simulink model "Controller_damping_cbf"  (R2026b)
settings: Solver=ode4  StopTime=Inf  FixedStep=1e-3
values from neighbouring files (symbols this model uses):
  cbf_damping_params = [cbf_p_ths; cbf_v_ths; cbf_v_0; cbf_gamma; cbf_d_max;                        cbf_w_lin; cbf_w_quad; plane_normal; plane_offset;                        cbf_latch_entry; cbf_zone_hyst; cbf_latch_alpha; cbf_clip_drift;                        cbf_tau_rate; cbf_dt; cbf_gamma_pos_scale]    [init_damping_cbf.m]
  Dn = 20 * ones(7,1)    [init_damping_cbf.m]
  H_0_cy = H_0_pr * H_pr_cy    [init_damping_cbf.m]
  H_home = getTransform(Franka_robot, q_home, 'panda_link8', 'panda_link0')    [init_damping_cbf.m]
  Kn = 0 * ones(7,1)    [init_damping_cbf.m]
  q_home = q_init    [init_damping_cbf.m]
  q_init = [0 0  0  -(2/4)*pi  0  pi/2  -pi/4]'    [init_damping_cbf.m]
undefined symbols (not defined in the file or in its folder): DiscIntNeverNeededParam, Fext_mag, T_final, X, Y, Z
libraries: sm_lib x162, nesl_utility x44, matrix_library x3, Robotics_lib x1
(part 8 of 12)

== matlab function Controller_damping_cbf/Dynamic Parameters/Mass Matrix1 ==
  data: q_state input; M output
function M = Franka_MassmMatrix(q_state)
% Author: TU Wien, ACIN Robotics group
% Optimized and generated from Maple
% hier wurden
% M_rot := Matrix(M_rot, shape=symmetric):
% M := simplify(Matrix( simplify(M_trans) + simplify(M_rot), shape=symmetric)):
% ausgefuehrt 

  M = zeros(7,7);

  t378 = q_state(6);
  t364 = sin(t378);
  t379 = q_state(5);
  t365 = sin(t379);
  t377 = q_state(7);
  t370 = cos(t377);
  t337 = 0.12763550042100000000e-2 * t370;
  t363 = sin(t377);
  t317 = 0.51602752476000000000e-3 * t363;
  t532 = t317 + 0.27219646194675000000e-1;
  t504 = t337 + t532;
  t308 = 0.13614453378240000000e-2 * t363;
  t267 = 0.5826996021941340000e-3 - t308;
  t357 = t370 ^ 2;
  t600 = 0.15804348732630080000e-2 * t357;
  t93 = t267 + (0.48418875570424600000e-2 * t363 + 0.55042935974400000000e-3) * t370 - t600;
  t45 = t365 * t93 + t504;
  t872 = t45 * t364;
  t371 = cos(t378);
  t871 = t45 * t371;
  t380 = q_state(4);
  t373 = cos(t380);
  t271 = 0.60149e-1 * t371 + 0.14117e-1 * t364;
  t372 = cos(t379);
  t638 = 0.10517e-1 * t365;
  t411 = -t271 * t372 + t638;
  t826 = 0.825e-1 + t411;
  t846 = t373 * t826;
  t381 = q_state(3);
  t367 = sin(t381);
  t474 = -0.10517e-1 * t370 - 0.4252e-2 * t363;
  t240 = -t474 + 0.88e-1;
  t639 = 0.61597e-1 * t364;
  t403 = t240 * t371 + t639;
  t812 = t365 * t403;
  t475 = 0.10517e-1 * t363 - 0.4252e-2 * t370;
  t844 = t372 * t475;
  t853 = (t844 - t812) * t367;
  t316 = 0.54835910640823200000e-3 * t363;
  t559 = 0.16724826617837780000e-2 * t370;
  t580 = 0.26431758938496000000e-1 * t364;
  t423 = t559 + t580;
  t311 = 0.10967182128164640000e-2 * t363;
  t553 = 0.33449653235675560000e-2 * t370;
  t442 = 0.11022068765350630000e-1 + t553;
  t183 = -t311 + t442;
  t358 = t371 ^ 2;
  t753 = t183 * t358;
  t642 = t316 - t423 - 0.44842466056464210000e-2 + t753;
  t250 = 0.12009367848960000000e-2 * t363 + 0.63347540234880000000e-1;
  t554 = 0.29704261916160000000e-2 * t370;
  t176 = t250 + t554;
  t351 = t363 ^ 2;
  t300 = 0.13297872941088000000e-4 * t351;
  t315 = 0.55042935974400000000e-3 * t363;
  t534 = -t315 - 0.57804776249276620000e-2;
  t333 = 0.24076459055801420000e-2 * t357;
  t592 = 0.79021743663150400000e-3 * t363;
  t721 = (-0.13614453378240000000e-2 + t592) * t370;
  t856 = t333 + t721;
  t833 = t534 + t856;
  t60 = -t300 + t833;
  t40 = -t364 * t60 + t176;
  t770 = t40 * t371;
  t870 = t642 - t770;
  t385 = -t365 * t475 - t372 * t403;
  t383 = q_state(1);
  t369 = sin(t383);
  t869 = t369 ^ 2;
  t376 = cos(t383);
  t868 = t376 ^ 2;
  t867 = t373 - 0.1e1;
  t313 = 0.68072266891200000000e-3 * t363;
  t222 = (0.24209437785212300000e-2 * t363 + 0.27521467987200000000e-3) * t370;
  t601 = 0.79021743663150400000e-3 * t357;
  t839 = t222 - t601;
  t413 = -0.29134980109706700000e-3 - t839;
  t87 = t313 + t413;
  t76 = t365 * t87;
  t834 = t315 + 0.32797153116247448000e-1 - t721;
  t481 = -t333 + t834;
  t62 = t300 + t481;
  t866 = t62 * t373;
  t65 = -0.825e-1 - t385;
  t865 = t65 * t373;
  t864 = t87 * t364;
  t74 = t87 * t371;
  t713 = t364 * t365;
  t863 = t87 * t713;
  t585 = 0.33449653235675560000e-2 * t363;
  t190 = 0.10967182128164639999e-2 * t370 + t585 + 0.18713819462921000000e-3;
  t144 = t190 * t365;
  t99 = 0.11357396418885000000e-1 - t144;
  t862 = t99 * t364;
  t673 = t300 + t315;
  t54 = (-0.69751885789075550000e-2 - t673 + t856) * t358;
  t710 = t364 * t371;
  t658 = t183 * t710;
  t817 = t658 - t54;
  t348 = 0.61597e-1 * t371;
  t836 = t240 * t364 - t348;
  t125 = 0.384e0 + t836;
  t366 = sin(t380);
  t848 = t125 * t366;
  t449 = 0.98827089590400000000e-3 * t363 + 0.52129746651620000000e-1;
  t556 = 0.24444132201840000000e-2 * t370;
  t198 = t449 + t556;
  t861 = t198 * t371;
  t182 = 0.59408523832320000000e-2 * t370 + 0.24018735697920000000e-2 * t363 + 0.12669508046976000000e0;
  t329 = 0.48152918111602840020e-2 * t357;
  t299 = 0.26595745882176000000e-4 * t351;
  t310 = 0.11008587194880000000e-2 * t363;
  t674 = t299 + t310;
  t508 = 0.11560955249855324002e-1 + t674;
  t590 = 0.15804348732630079999e-2 * t363;
  t722 = (-0.27228906756480000000e-2 + t590) * t370;
  t788 = t722 + t329 - t508;
  t645 = t364 * t788 - t182;
  t860 = t371 * t645;
  t334 = 0.15804348732630079999e-2 * t357;
  t521 = -t334 + t267;
  t724 = (0.48418875570424600020e-2 * t363 + 0.55042935974400000000e-3) * t370;
  t488 = t724 + t521;
  t859 = t488 * t365;
  t705 = t365 * t372;
  t560 = 0.14820000000000000000e-2 * t370;
  t287 = t364 * t560;
  t587 = 0.23920000000000000000e-2 * t363;
  t716 = (0.68200e-3 + t587) * t364;
  t451 = 0.17120000000000000000e-2 * t357 + 0.14600000000000000000e-2;
  t714 = t363 * t370;
  t517 = 0.49780000000000000000e-2 * t714;
  t394 = -t451 + t517;
  t762 = t394 * t371;
  t784 = t762 - t716 - t287 - 0.42340e-2;
  t858 = t705 * t784;
  t133 = t504 * t371;
  t824 = 0.11357396418885000000e-1 * t364 - 0.24178658687700000000e-2;
  t797 = t133 + t824;
  t79 = t797 * t372;
  t359 = t372 ^ 2;
  t427 = 0.10967182128164640000e-2 * t370 + t585;
  t189 = t427 + 0.18713819462921000000e-3;
  t748 = t189 * t364;
  t606 = t748 + 0.5437511053345940e-2;
  t849 = t93 * t371;
  t815 = t849 - t606;
  t857 = t815 * t359;
  t598 = 0.24890000000000000000e-2 * t357;
  t416 = t598 + 0.85600000000000000000e-3 * t714;
  t38 = t849 - t748 - 0.54375110533459400000e-2;
  t185 = -0.59408523832320000000e-2 * t363 + 0.47796540830203740000e-1 + 0.24018735697920000000e-2 * t370;
  t752 = t185 * t365;
  t540 = t752 + 0.27752814537092170000e0;
  t854 = -t371 * t99 + t540;
  t352 = t364 ^ 2;
  t284 = t370 * t592;
  t495 = t284 + 0.24209437785212300000e-2 * t357;
  t759 = (t495 + 0.1194710953979893e-2) * t352;
  t852 = 0.25054324779447817000e-1 + t759;
  t382 = q_state(2);
  t375 = cos(t382);
  t850 = t375 ^ 2;
  t847 = t826 * t366;
  t256 = 0.56786982094425000000e-2 * t364 - 0.12089329343850000000e-2;
  t229 = t256 * t373;
  t845 = t366 * t371;
  t374 = cos(t381);
  t700 = t366 * t374;
  t694 = t367 * t374;
  t688 = t371 * t373;
  t687 = t371 * t374;
  t683 = t373 * t374;
  t468 = 0.39252e-1 * t367 - 0.27518e-1 * t374;
  t843 = t375 * t468;
  t581 = 0.21751134959804000000e-1 * t364;
  t842 = (t581 - 0.46305794820080000000e-2 + t861) * t372;
  t672 = 0.31608697465260159998e-2 * t357 + 0.27228906756480000000e-2 * t363;
  t461 = (0.96837751140849200040e-2 * t363 + 0.11008587194880000000e-2) * t370 - t672 + 0.11653992043882680000e-2;
  t72 = t461 * t371;
  t804 = t504 * t364;
  t158 = t416 + 0.28220000000000000000e-2;
  t763 = t158 * t358;
  t389 = t763 + t416 - 0.27050000000000000000e-2;
  t307 = 0.14820000000000000000e-2 * t363;
  t558 = 0.23920000000000000000e-2 * t370;
  t491 = -t307 + t558;
  t657 = (0.21800000000000000000e-3 + t491) * t710;
  t841 = (-t657 + t389) * t359;
  t332 = 0.24076459055801420010e-2 * t357;
  t593 = 0.79021743663150399997e-3 * t363;
  t838 = -(-0.13614453378240000000e-2 + t593) * t370 - t332 + t673;
  t53 = (0.69751885789075550010e-2 + t838) * t358;
  t285 = t370 * t593;
  t837 = t285 + 0.25022978729410880010e-2 * t357;
  t298 = 0.81354094419858000000e-4 * t351;
  t318 = 0.11947109539798930000e-2 * t352;
  t670 = t318 - t298;
  t579 = 0.61597000000000000000e-1 * t364;
  t216 = 0.10517000000000000000e-1 * t363 - 0.42520000000000000000e-2 * t370;
  t197 = 0.10517000000000000000e-1 * t370 + 0.42520000000000000000e-2 * t363 + 0.88000000000000000000e-1;
  t742 = t197 * t371;
  t681 = -t216 * t365 - t372 * t742;
  t835 = -t372 * t579 + t681 + 0.82500000000000000000e-1;
  t473 = 0.60149e-1 * t364 - 0.14117e-1 * t371;
  t234 = t473 + 0.384e0;
  t728 = t234 * t373;
  t832 = t366 * t411 - t728;
  t342 = 0.13297872941088e-4 * t351;
  t67 = -t342 + t833;
  t57 = t67 * t364;
  t831 = t57 - 0.1e1 * t176;
  t415 = 0.49780000000000000000e-2 * t357 + 0.17120000000000000000e-2 * t714;
  t167 = 0.5644000000000000000e-2 + t415;
  t122 = t167 * t358;
  t492 = -0.47840000000000000000e-2 * t370 + 0.29640000000000000000e-2 * t363;
  t210 = 0.43600e-3 - t492;
  t126 = t210 * t710;
  t680 = t122 - t126;
  t830 = 0.31784000000000000000e-1 + t680 - 0.1e1 * t416;
  t314 = 0.63817750210500000000e-3 * t363;
  t567 = 0.25801376238000000000e-3 * t370;
  t445 = 0.55993270925625000000e-2 + t567;
  t191 = -t314 + t445;
  t676 = t284 + 0.25022978729410880000e-2 * t357;
  t84 = 0.25565950283854690000e-2 - t676 + t670;
  t33 = t84 + t817;
  t829 = t33 * t365 - 0.1e1 * t191;
  t828 = -0.1e1 * t185 - 0.1e1 * t190 * t371;
  t368 = sin(t382);
  t171 = t368 * t468 + 0.249498e0 * t375;
  t572 = 0.21751134959804000000e-1 * t366;
  t825 = t133 - 0.24178658687700000000e-2;
  t823 = 0.56786982094425000000e-2 * t371 + 0.12908973617152500000e-1;
  t259 = 0.11357396418885000000e-1 * t366 - 0.52863517876992000000e-1;
  t309 = 0.12763550042100000000e-2 * t363;
  t566 = 0.51602752476000000000e-3 * t370;
  t444 = 0.11198654185125000000e-1 + t566;
  t175 = -t309 + t444;
  t756 = t175 * t365;
  t822 = (-t366 * t504 + t182) * t364 + 0.16910953236199946500e0 + t259 * t371 + (-0.1e1 * t756 + t79 - 0.31476782229750000000e-1) * t373 - 0.10663433246449500000e0 * t366;
  t589 = 0.15804348732630080000e-2 * t363;
  t813 = t364 * ((-0.27228906756480000000e-2 + t589) * t370 + 0.48152918111602840000e-2 * t357 - t674 - 0.11560955249855324000e-1);
  t37 = (-t182 + t813) * t371;
  t552 = 0.66899306471351120000e-2 * t370;
  t424 = -0.21934364256329280000e-2 * t363 + t552;
  t319 = 0.52863517876992000000e-1 * t364;
  t453 = 0.8968493211292842000e-2 + t553;
  t437 = t319 + t453;
  t408 = -(t424 + 0.22044137530701260000e-1) * t358 - t311 + t437;
  t97 = t189 * t365 - 0.11357396418885000000e-1;
  t771 = t371 * t97;
  t819 = (t37 - t408) * t372 + t771;
  t173 = t271 * t365 + 0.10517e-1 * t372;
  t406 = t173 * t367;
  t215 = t234 * t366;
  t207 = -0.825e-1 + t215;
  t803 = t207 + t846;
  t818 = t374 * t803 + t406;
  t263 = 0.25801376238000000000e-3 * t363 + 0.13609823097337500000e-1;
  t564 = 0.63817750210500000000e-3 * t370;
  t199 = t263 + t564;
  t739 = t199 * t373;
  t293 = 0.88e-1 * t364 + 0.384e0;
  t814 = t293 * t367;
  t338 = 0.98827089590400000000e-3 * t370;
  t448 = 0.24444132201840000000e-2 * t363 - 0.21447119530300000000e-1;
  t800 = -t338 + t448;
  t807 = t800 * t367;
  t628 = 0.345563e0 * t373;
  t472 = 0.41065e-1 * t365 + 0.11953e-1 * t372;
  t235 = t472 + 0.825e-1;
  t727 = t235 * t366;
  t502 = -t628 + t727;
  t806 = (t502 - 0.316e0) * t375;
  t805 = (-0.41065e-1 * t372 + 0.11953e-1 * t365) * t367;
  t345 = 0.345563e0 * t366;
  t290 = -0.825e-1 + t345;
  t726 = t235 * t373;
  t524 = t290 + t726;
  t105 = t524 * t374;
  t150 = t199 * t371;
  t802 = t256 + t150;
  t277 = t307 - 0.829200e-2;
  t659 = t167 * t710;
  t732 = t210 * t358;
  t801 = t277 - t558 + t659 + t732;
  t426 = -t560 - t587;
  t730 = (-t426 + 0.68200e-3) * t371;
  t799 = t394 * t364 + t730 - 0.45800e-3;
  t798 = t300 - 0.1e1 * t333 - 0.26431758938496000000e-1 * t371 + t834;
  t796 = 0.46331267916800000000e-2 - t837;
  t794 = 0.53124178491565338000e0 + t673 + 0.2251687828321245e-2 * t359;
  t618 = 0.7735484874e-2 * t370;
  t793 = 0.3127439544e-2 * t363 + t618;
  t660 = t158 * t710;
  t211 = 0.21800e-3 + t491;
  t731 = t211 * t358;
  t791 = -t660 - t731;
  t460 = -t670 + t837;
  t312 = 0.10967182128164639999e-2 * t363;
  t184 = -t312 + t442;
  t662 = t184 * t710;
  t790 = t662 - t460 + 0.48082828567067140000e-2;
  t484 = -t722 + 0.13950377157815110002e-1 + t674;
  t392 = -t739 + t199;
  t164 = t333 + t284 - 0.9457555763200000000e-3;
  t787 = t164 * t358 - t658;
  t565 = 0.54835910640823200000e-3 * t370;
  t588 = 0.16724826617837780000e-2 * t363;
  t430 = t565 + t588;
  t202 = t430 + 0.9356909731460500000e-4;
  t737 = t202 * t371;
  t786 = t864 - 0.1e1 * t737;
  t341 = 0.4815291811160284002e-2 * t357;
  t678 = t722 + t341;
  t785 = -0.1e1 * t319 + ((-t508 + t678) * t364 - t182) * t371;
  t282 = t370 * t589;
  t336 = 0.13614453378240000000e-2 * t370;
  t671 = t315 + t336;
  t755 = (0.60427308755286430000e-2 + t671) * t352;
  t783 = t282 + t756 - 0.1e1 * t755;
  t782 = -t716 - 0.15700e-2;
  t489 = -t316 + t559;
  t186 = t489 + 0.44842466056464210000e-2;
  t326 = 0.56786982094425000000e-2 * t366;
  t528 = t326 - 0.21751134959804000000e-1;
  t545 = 0.26431758938496000000e-1 * t373;
  t573 = 0.12089329343850000000e-2 * t366;
  t780 = (t186 * t373 + (-0.1e1 * t528 + t545) * t364 + t573 - 0.46305794820080000000e-2) * t372 + t852 * t366;
  t156 = -0.85600000000000000000e-3 * t357 + 0.24890000000000000000e-2 * t714 - 0.73000000000000000000e-3;
  t709 = t364 * t372;
  t779 = -t156 * t709 - 0.86410e-2;
  t734 = (0.6042730875528643e-2 + t671) * t352;
  t777 = t734 + 0.65337013765020712700e0;
  t283 = t370 * t590;
  t353 = t365 ^ 2;
  t320 = 0.22516878283212450000e-2 * t353;
  t531 = t320 - 0.54359965714773641100e0;
  t754 = t182 * t364;
  t775 = 0.48418875570424600020e-2 * t357 + (t184 * t364 + 0.52863517876992000000e-1) * t371 + t283 + t531 - t754 - t755 + t756;
  t774 = -t176 * t372 + 0.56786982094425000000e-2;
  t773 = t870 * t365;
  t86 = t334 - t724 - 0.58269960219413400000e-3 + t308;
  t772 = t371 * t86;
  t537 = t197 * t364 + 0.38400000000000000000e0;
  t767 = (-t348 + t537) * t366;
  t766 = (-t199 + 0.21751134959804000000e-1 * t372) * t373;
  t523 = 0.6029433002587555e-2 + t671;
  t765 = (t300 + t523) * t358;
  t764 = (-0.99560000000000000000e-2 * t714 + 0.34240000000000000000e-2 * t357 + 0.29200000000000000000e-2) * t371;
  t121 = (0.2489553776598930000e-3 + t495) * t358;
  t758 = t800 * t365;
  t757 = t800 * t373;
  t137 = t176 * t366;
  t306 = 0.21934364256329279998e-2 * t363;
  t441 = 0.22044137530701260000e-1 + t552;
  t181 = -t306 + t441;
  t134 = t181 * t358;
  t187 = 0.69884864518486430000e-2 + t671;
  t751 = t187 * t373;
  t303 = 0.29704261916160000000e-2 * t363;
  t561 = 0.12009367848960000000e-2 * t370;
  t443 = 0.23898270415101870000e-1 + t561;
  t188 = -t303 + t443;
  t750 = t188 * t365;
  t749 = t188 * t373;
  t746 = t191 * t365;
  t745 = t191 * t366;
  t323 = 0.82500000000000000002e-1 * t366;
  t194 = t323 - 0.31600000000000000000e0 * t373 - 0.38400000000000000000e0;
  t744 = t194 * t371;
  t196 = 0.48888264403680000000e-2 * t370 + 0.19765417918080000000e-2 * t363 + 0.10425949330324000000e0;
  t743 = t196 * t364;
  t147 = t198 * t364;
  t741 = t198 * t373;
  t740 = t199 * t364;
  t149 = t199 * t366;
  t154 = t202 * t364;
  t738 = t202 * t365;
  t736 = t202 * t374;
  t490 = -t311 + t553;
  t203 = 0.11022068765350630e-1 + t490;
  t735 = t203 * t358;
  t205 = 0.187138194629210e-3 + t427;
  t733 = t205 * t365;
  t563 = 0.74100000000000000000e-3 * t370;
  t591 = 0.11960000000000000000e-2 * t363;
  t429 = -t563 - t591;
  t213 = -t429 + 0.34100e-3;
  t729 = t213 * t371;
  t723 = (0.68200000000000000000e-3 + t587) * t364;
  t254 = t314 - 0.55993270925625000000e-2;
  t720 = t254 * t366;
  t264 = 0.11198654185125000000e-1 - t309;
  t719 = t264 * t365;
  t718 = (0.4841887557042460002e-2 * t363 + 0.55042935974400000000e-3) * t370;
  t715 = t353 * t364;
  t712 = t364 * t366;
  t711 = t364 * t367;
  t708 = t364 * t373;
  t707 = t365 * t366;
  t706 = t365 * t371;
  t704 = t365 * t375;
  t703 = t366 * t367;
  t702 = t366 * t372;
  t701 = t366 * t373;
  t699 = t366 * t375;
  t698 = t367 * t365;
  t697 = t367 * t369;
  t696 = t367 * t372;
  t695 = t367 * t373;
  t692 = t367 * t376;
  t691 = t368 * t369;
  t690 = t368 * t376;
  t689 = t369 * t374;
  t686 = t371 * t375;
  t685 = t372 * t373;
  t684 = t372 * t375;
  t682 = t373 * t375;
  t656 = t211 * t710;
  t679 = t656 - t763;
  t344 = 0.3507900e-3 * t365;
  t288 = -0.925496e-3 - t344;
  t677 = t288 * t373 + t344;
  t647 = 0.825e-1 * t374;
  t295 = t368 * t647;
  t649 = 0.825e-1 * t366;
  t675 = -t375 * t649 - t295;
  t669 = t762 - 0.1e1 * t287;
  t666 = t373 * t759;
  t180 = -0.21934364256329279999e-2 * t363 + t441;
  t665 = t180 * t710;
  t664 = t181 * t710;
  t111 = t183 * t708;
  t663 = t374 * t753;
  t661 = t359 * t699;
  t655 = t365 * t699;
  t653 = t183 * t712;
  t652 = t366 * t686;
  t350 = 0.316e0 * t368;
  t651 = t368 * t649 + t647 * t682 - t350;
  t648 = 0.825e-1 * t367;
  t643 = -0.7850e-3 + (-0.34100e-3 - t591) * t364;
  t637 = 0.27454e-1 * t367;
  t631 = 0.249498e0 * t368;
  t630 = 0.735522e0 * t371;
  t623 = 0.384e0 * t699 * t374 + t651;
  t622 = 0.8676525e-3 * t365;
  t620 = 0.3127439544e-2 * t365;
  t619 = 0.7735484874e-2 * t365;
  t617 = 0.3127439544e-2 * t373;
  t616 = 0.7735484874e-2 * t373;
  t615 = 0.3127439544e-2 * t370;
  t614 = 0.735522e0 * t700;
  t613 = 0.6381775021050e-3 * t366;
  t612 = 0.2580137623800e-3 * t367;
  t611 = 0.6381775021050e-3 * t367;
  t609 = t728 - t847;
  t438 = t312 - t453;
  t604 = t438 * t365 + 0.3288975154738540000e-2;
  t603 = t79 - 0.80863245317250000000e-1;
  t602 = 0.23894219079597860000e-2 * t352;
  t596 = 0.50045957458821760020e-2 * t357;
  t595 = 0.28220000000000000000e-2 * t358;
  t594 = 0.74100000000000000000e-3 * t363;
  t586 = 0.31608697465260159998e-2 * t363;
  t584 = 0.66899306471351120000e-2 * t363;
  t583 = 0.49096519673609460000e-2 * t364;
  t578 = 0.88000000000000000000e-1 * t364;
  t577 = 0.24178658687700000000e-2 * t365;
  t576 = 0.49096519673609460000e-2 * t365;
  t575 = 0.26431758938496000000e-1 * t365;
  t574 = 0.54835910640823200000e-3 * t366;
  t570 = 0.31600000000000000000e0 * t366;
  t569 = 0.16724826617837780000e-2 * t367;
  t568 = 0.46305794820080000000e-2 * t367;
  t562 = 0.11960000000000000000e-2 * t370;
  t555 = 0.29640000000000000000e-2 * t370;
  t551 = 0.16724826617837780000e-2 * t371;
  t550 = 0.11357396418885000000e-1 * t371;
  t549 = 0.54835910640823200000e-3 * t373;
  t548 = 0.16724826617837780000e-2 * t373;
  t547 = 0.49096519673609460000e-2 * t373;
  t546 = 0.21751134959804000000e-1 * t373;
  t543 = 0.21751134959804000000e-1 * t371;
  t542 = t364 * t612;
  t541 = t364 * t611;
  t538 = t190 * t364 + 0.54375110533459400000e-2;
  t536 = t287 + 0.42340000000000000000e-2;
  t530 = 0.43502269919608000000e-1 * t366 - 0.11357396418885000000e-1;
  t529 = -t326 + 0.26431758938496000000e-1;
  t527 = 0.12089329343850000000e-2 * t867;
  t343 = 0.13297872941088e-4 * t357;
  t526 = -t343 - 0.11947109539798930000e-2;
  t525 = 0.23898270415101870000e-1 - t303;
  t522 = t540 + t872;
  t470 = -0.104419e0 * t366 - 0.5317e-1 * t373;
  t236 = -t470 - 0.825e-1;
  t520 = t236 * t374 - t637;
  t516 = t365 * t581;
  t515 = t364 * t549;
  t514 = t364 * t548;
  t513 = 0.49096519673609460000e-2 * t845;
  t512 = t364 * t563;
  t511 = t372 * t547;
  t503 = 0.48082828567067140000e-2 - t676;
  t501 = -0.52863517876992000000e-1 * t371 + t754;
  t425 = -0.21934364256329279998e-2 * t370 - t584;
  t201 = -t425 + 0.3742763892584200000e-3;
  t499 = -t201 * t364 - 0.10875022106691880000e-1;
  t498 = -0.56786982094425000000e-2 + t738;
  t266 = 0.9356909731460500000e-4 + t588;
  t496 = t266 + t565;
  t494 = -t284 - t598;
  t493 = -t285 - 0.24209437785212300010e-2 * t357;
  t487 = t504 + t859;
  t486 = -t565 - 0.1e1 * t266;
  t479 = -t298 + t503;
  t217 = -0.41065000000000000000e-1 * t372 + 0.11953000000000000000e-1 * t365;
  t478 = t217 * t374 + t367 * t524;
  t469 = -0.104419e0 * t373 + 0.5317e-1 * t366;
  t467 = -0.39252e-1 * t374 - 0.27518e-1 * t367;
  t466 = t496 * t365;
  t464 = (0.13297872941088000000e-4 * t357 - t670 - t817 - 0.46331267916800000000e-2) * t359 + t38 * t705 + t501;
  t463 = -0.1e1 * t318 - t479;
  t459 = t54 - t84;
  t328 = 0.48418875570424600000e-2 * t357;
  t456 = -t79 + t658 - t121 + (t494 + 0.175156065026714e-3) * t359 + t320 + t328 - 0.37693495392476464200e0;
  t253 = -t313 + 0.29134980109706700000e-3;
  t455 = -0.1e1 * t222 + t601 - 0.1e1 * t253;
  t454 = -0.5437511053345940e-2 * t365 - 0.24178658687700000000e-2;
  t260 = 0.56786982094425000000e-2 * t867;
  t446 = -0.54375110533459400000e-2 * t365 - 0.24178658687700000000e-2;
  t232 = 0.16724826617837780000e-2 * t374 + 0.988270895904e-3 * t367;
  t440 = 0.2444413220184e-2 * t367 + 0.54835910640823200000e-3 * t374;
  t439 = 0.7902174366315040000e-3 * t357 + t313 - 0.2913498010970670000e-3;
  t436 = (t469 - 0.316e0) * t375;
  t433 = 0.48888264403680000000e-2 * t363 - 0.19765417918080000000e-2 * t370 - 0.42894239060600000000e-1;
  t431 = -0.1e1 * t338 + t448;
  t428 = t562 - t594;
  t422 = -t546 + t326;
  t421 = t134 + t438;
  t231 = t263 * t366;
  t324 = 0.82500000000000000000e-1 * t366;
  t257 = t324 - 0.38400000000000000000e0;
  t420 = t257 * t618 + t231 - t250;
  t297 = 0.16270818883971600000e-3 * t351;
  t419 = t283 + t297 - 0.51131900567709380000e-2 - t602;
  t417 = -0.1e1 * t303 - t864 + t443;
  t172 = -t631 + t843;
  t409 = t366 * t472 - t628;
  t206 = -t430 - 0.93569097314605e-4;
  t402 = t423 + 0.4484246605646421e-2;
  t258 = -t324 + 0.31600000000000000000e0;
  t401 = t258 * t618 + t449;
  t400 = t430 + 0.935690973146050000e-4;
  t398 = -0.25527100084200000000e-2 * t370 - 0.10320550495200000000e-2 * t363 - 0.54439292389350000000e-1;
  t397 = 0.11881704766464000000e-1 * t370 + 0.48037471395840000000e-2 * t363 + 0.25339016093952000000e0;
  t396 = -t415 + 0.5410000000000000000e-2;
  t393 = -t415 + 0.33106000000000000000e-1;
  t390 = t602 + t665 - 0.1e1 * t283 - 0.1e1 * t297 - t596;
  t388 = t763 + t393;
  t386 = -t186 + 0.46305794820080000000e-2 * t373 - t573;
  t384 = -t125 * t373 + t366 * t385;
  t361 = t374 ^ 2;
  t360 = t373 ^ 2;
  t355 = t367 ^ 2;
  t354 = t366 ^ 2;
  t340 = 0.21751134959804000000e-1 * t374;
  t327 = 0.54835910640823200000e-3 * t367;
  t322 = 0.56786982094425000000e-2 * t365;
  t321 = 0.17515606502671400000e-3 * t353;
  t289 = t622 - 0.374176e-3;
  t286 = t367 * t567;
  t278 = 0.414600e-2 - t594;
  t276 = 0.47840000000000000000e-2 * t363 + 0.136400e-2;
  t274 = -0.2872e-1 * t375 - 0.3141e-2 * t368;
  t269 = t289 * t373;
  t261 = -0.82500000000000000002e-1 + t570;
  t255 = 0.38400000000000000000e0 + t578;
  t230 = t449 * t367;
  t228 = t256 * t366;
  t195 = 0.38400000000000000000e0 * t373 - t323 + 0.31600000000000000000e0;
  t193 = -t260 - 0.26431758938496000000e-1 * t366;
  t163 = t332 + t285 - 0.9457555763200000010e-3;
  t155 = t202 * t372;
  t145 = t191 * t373;
  t140 = t186 * t366;
  t129 = t433 * t365;
  t120 = t202 * t688;
  t106 = t154 + 0.6624110552949070e-2;
  t103 = -t194 + t578;
  t101 = -t190 + 0.11357396418885000000e-1 * t365;
  t90 = -t804 + t550 - 0.28391278634449500000e0;
  t89 = -0.61597000000000000000e-1 * t371 + t537;
  t77 = t87 * t374;
  t71 = -t489 * t364 + (-0.680722668912e-3 * t370 - 0.275214679872e-3 * t363 - 0.49096519673609460000e-2) * t371;
  t70 = t87 * t708;
  t68 = -t805 + t105;
  t51 = t844 + (-t639 - t742) * t365;
  t49 = -t372 * t639 + t681 + 0.825e-1;
  t42 = t371 * t496 - t864;
  t36 = -t656 + t389;
  t26 = 0.155920e-1 + t801 * t372 + t799 * t365;
  t25 = t429 * t372 + (t371 * t428 - t583 - t793 * (t293 - t348)) * t365 + (0.7735484874e-2 * t363 - t615) * (-(-0.384e0 * t371 + 0.61597e-1) * t372 + 0.825e-1 * t364);
  t24 = t798 * t372 + t74 * t365 - t150 + (t466 - t774) * t364;
  t20 = -t773 + (t188 + t737 - t864) * t372;
  t19 = ((t293 * t793 - t371 * t489 + t583) * t372 + (0.28244044800000000000e0 * t216 * t371 - t430) * t365) * t366 - 0.606805650e-1 * t474 * t867 * t372 + (-0.1e1 * t547 + 0.735522e0 * t677 * t370 + 0.735522e0 * (t269 - 0.1e1 * t622) * t363) * t371 - t370 * t514 + t363 * t515;
  t18 = ((t176 * t364 + t798) * t365 + (-0.1e1 * t154 - t74) * t372) * t366 + ((-0.1e1 * t564 - 0.1e1 * t263 + t739) * t364 - t260 * t371) * t365 - t70 + t120;
  t13 = (t466 * t371 - t863 + (t371 * t831 + t642) * t372) * t366 + t358 * t751 + (t372 * t392 + t111) * t371 + (-t260 * t364 + t527) * t372 + t666 + 0.25054324779447817000e-1 * t373 + ((t561 + t525) * t366 + (-0.1e1 * t254 + t567) * t373 - 0.1e1 * t567 + t254) * t365;
  t12 = (((t255 * t616 - t371 * t548 - 0.63817750210500000002e-3 * t366 + 0.24444132201840000000e-2) * t372 + (-0.4252e-2 * t195 * t365 + 0.92549600000000000000e-3 * t366) * t630 - t365 * t549) * t370 + ((t255 * t617 + t371 * t549 - 0.25801376238000000001e-3 * t366 + 0.98827089590400000000e-3) * t372 + (t195 * t638 + 0.37417600000000000000e-3 * t366) * t630 - t365 * t548) * t363 + t513) * t367 + (((-0.3127439544e-2 * t744 + 0.54835910640823200000e-3) * t372 - t365 * t551 + t103 * t619) * t370 + ((0.7735484874e-2 * t744 + 0.16724826617837780000e-2) * t372 + 0.54835910640823200000e-3 * t706 + t103 * t620) * t363) * t374 + ((-t363 * t574 + t366 * t559 + t511) * t367 + ((-0.3127439544e-2 * t261 - 0.25801376238000000001e-3 * t373) * t370 + (0.7735484874e-2 * t261 + 0.63817750210500000002e-3 * t373) * t363 + t576) * t374) * t364;
  t11 = ((t33 * t372 - t802) * t365 + t38 * t359 - 0.1e1 * t191 * t372 + t74 + t154 + 0.66241105529490700000e-2) * t366 + (-t773 + (t417 + t737) * t372 - 0.1644487577369270e-2) * t373;
  t10 = (((-t198 * t372 - 0.56786982094425000000e-2) * t373 + t420 * t372 - t572 - t498) * t364 + (t766 + t529 * t372 - t76 + (0.82500000000000000000e-1 - t570) * t618 - t449 * t366 + t263) * t371 - t62 * t372) * t374 + (((t176 * t365 - t155) * t373 + t401 * t365) * t364 + ((-t372 * t87 - t575) * t373 + t528 * t365) * t371 + t365 * t866 + ((-0.1e1 * t263 * t365 + t455) * t364 + t486 * t371) * t366) * t367;
  t9 = ((((t232 * t373 - 0.1e1 * t366 * t612 + 0.1200936784896e-2 * t367) * t371 + t327 + (-0.1e1 * t293 * t616 + t613 - 0.2444413220184e-2) * t374) * t372 + (t288 * t614 + (-0.1e1 * t569 + (0.1200936784896e-2 * t373 + 0.988270895904e-3) * t374) * t365) * t371 + (t365 * t440 - 0.1e1 * t542) * t373 + (-0.1e1 * t232 * t364 - 0.1e1 * t365 * t611) * t366 + t619 * t814 + t542) * t370 + (((-0.5483591064082320000e-3 * t683 + (-0.2444413220184e-2 * t373 + t613 - 0.2970426191616e-2) * t367) * t371 + 0.2580137623800e-3 * t700 + t569 + (-0.1e1 * t293 * t617 - 0.988270895904e-3) * t374) * t372 + (t289 * t614 + (t327 + (-0.2970426191616e-2 * t373 - 0.2444413220184e-2) * t374) * t365) * t371 + (t232 * t365 + t541) * t373 + (t364 * t440 - 0.1e1 * t365 * t612) * t366 + t620 * t814 - 0.1e1 * t541) * t363 - 0.1e1 * t364 * t374 * t511 - 0.1e1 * t374 * t513 + t576 * t711) * t368 + (0.49096519673609460000e-2 * t364 * t702 - 0.49096519673609460000e-2 * t688 + ((0.7735484874e-2 * t293 * t366 + 0.6381775021050e-3 * t867) * t372 + (-0.1632768e-2 * t707 + t677) * t630 - 0.1e1 * t365 * t574 - 0.1e1 * t551 * t702 - 0.1e1 * t514) * t370 + (((0.3127439544e-2 * t293 + 0.5483591064082320000e-3 * t371) * t366 + 0.2580137623800e-3 * t373 - 0.2580137623800e-3) * t372 + (t269 + (0.4038528e-2 * t366 - 0.8676525e-3) * t365) * t630 + t515 - 0.16724826617837780000e-2 * t707) * t363) * t375;
  t8 = ((t183 * t685 + (-t336 - 0.1e1 * t315 - 0.69884864518486430000e-2) * t366) * t358 + ((t231 - t401) * t372 - 0.1e1 * t653 + (t372 * t831 + t738) * t373) * t371 + (t258 * t615 - t448 - t70 + t720 + t749) * t365 - t780) * t367 + t365 * t663 + (-t155 + (t420 + t57 - t741) * t365) * t687 + ((t257 * t615 - t525 - t720 + t757 + t864) * t372 + ((-t529 - t546) * t364 + t386) * t365) * t374;
  t7 = (((-t202 * t367 + (-t176 * t373 + t149 - t198) * t374) * t365 + (-0.56786982094425000000e-2 * t367 + (-t198 * t367 + t374 * t400) * t372) * t373 + ((t199 * t372 - 0.21751134959804000000e-1) * t367 + (t253 + t839) * t374) * t366 + t774 * t367) * t364 + ((-t367 * t87 + t340) * t371 + ((t545 - t326) * t371 - t866) * t374) * t365 + ((t766 + (-t198 - 0.56786982094425000000e-2 * t372) * t366 + 0.26431758938496000000e-1 * t372 + t199) * t367 + (t496 * t366 + (-0.1e1 * t222 + t439) * t685) * t374) * t371 - t62 * t696) * t368 + t375 * ((t137 - t392) * t365 - t87 * t373 - t400 * t702) * t364 + (t193 * t371 + t366 * t62) * t704 + (t202 * t373 + (t222 - t439) * t702) * t686;
  t6 = (((-t137 - t739) * t371 - t140 - t229) * t365 + ((-0.1e1 * t188 + t786) * t372 + 0.1644487577369270e-2 + (t753 + (t60 * t371 - 0.26431758938496000000e-1) * t364) * t365) * t366) * t367 + ((-0.1e1 * t765 + t463) * t359 + ((-0.1e1 * t198 * t366 - t739 + t45) * t371 - t606 * t365 - t229 + (0.11357396418885000000e-1 - t572) * t364 + 0.46305794820080000000e-2 * t366 - 0.24178658687700000000e-2) * t372 + (-0.1e1 * t164 * t353 - 0.1e1 * t343 - 0.1194710953979893e-2) * t358 + (t183 * t715 - 0.1e1 * t326 + 0.52863517876992000000e-1) * t371 - 0.1e1 * t320 + (-0.1e1 * t800 * t366 + t145 - t175) * t365 + (-t182 + t149) * t364 + 0.29682175996164750000e0 * t366 - t777) * t374 + ((t372 * t829 + t106 + t74 + t857) * t367 + (-t147 - 0.50330438027992300000e0 + t543) * t374) * t373;
  t5 = ((t187 * t700 + (-0.1e1 * t372 * t683 + t698) * t183) * t358 + t683 * t863 + ((t486 * t372 + (t57 - 0.1e1 * t741 + t149 - 0.1e1 * t554 - 0.1e1 * t250) * t365) * t371 + (t364 * t455 - 0.1e1 * t525 - 0.1e1 * t561 + t745 + t757) * t372 + (t422 - 0.26431758938496000000e-1) * t713 + t386 * t365) * t367 + (((-0.1e1 * t149 + t198) * t372 + t653 + (((-0.1e1 * t333 - 0.1e1 * t721 + t342 - 0.1e1 * t534) * t364 + t176) * t372 - 0.1e1 * t738) * t373) * t371 + (-0.1e1 * t749 + t745 + t431) * t365 + t780) * t374) * t368 + ((t67 * t712 - 0.1e1 * t137 + t392) * t372 + t111 + t202 * t707) * t686 + (t193 * t364 - 0.1e1 * t140 + t527) * t684 - t655 * t864 + (t188 * t366 + t145 - 0.1e1 * t191) * t704 + 0.25054324779447817000e-1 * t682 + ((t183 * t702 + t751) * t358 + t666) * t375;
  t4 = (-0.36044563611157510600e0 + (((0.22044137530701260e-1 + t424) * t358 + t37 - 0.1e1 * t319 - 0.8968493211292842e-2 - 0.1e1 * t490) * t372 + (-0.11357396418885000000e-1 + t733) * t371 + t522) * t360 + (-0.1e1 * t842 - 0.1e1 * t740 - 0.1e1 * t758 + t823) * t373 + (-0.1e1 * t735 + (-0.1e1 * t149 + t40) * t371 - 0.1e1 * t228 - 0.1e1 * t316 + t402) * t372 + (t206 * t365 + 0.56786982094425000000e-2) * t371 + (t76 - 0.1e1 * t199) * t364 - 0.1e1 * t750 + (((-0.1e1 * t203 * t710 + t54 + t463) * t359 + (t871 + (-0.1e1 * t733 + 0.11357396418885000000e-1) * t364 + t454) * t372 + t121 + (-0.1e1 * t203 * t364 - 0.52863517876992000000e-1) * t371 + t734 + t754 - 0.1e1 * t320 - 0.1e1 * t756 - 0.1e1 * t328 - 0.1e1 * t282 + 0.54359965714773641100e0) * t373 - 0.1e1 * t543 + t746 + t147 + 0.58416762559717300000e0) * t366) * t367 + ((t206 * t371 - 0.1e1 * t188 + t864) * t372 + 0.1644487577369270e-2 + (t316 - 0.1e1 * t402 + t735 - t770) * t365) * t683 + ((t199 * t365 - t87) * t366 - 0.1e1 * t198 * t365) * t687 + ((t205 * t364 - t849 + 0.5437511053345940e-2) * t359 + (t206 + t322) * t364 - 0.12089329343850000000e-2 * t365 - 0.6624110552949070e-2) * t700 + (((-0.1e1 * t314 + t445) * t366 + (-0.1e1 * t203 * t710 + t459) * t707 + t431) * t372 - 0.1e1 * t516 + 0.46305794820080000000e-2 * t365 - 0.13297019103287584000e-1) * t374;
  t3 = t815 * t661 + (t366 * t829 + t373 * t417 + t120) * t684 + (-0.1e1 * t149 * t371 - t870 * t373 - 0.1e1 * t228) * t704 + t87 * t652 - 0.1644487577369270e-2 * t682 + t106 * t699 + (-t683 * t857 + ((-0.1e1 * t111 * t687 - 0.1e1 * t205 * t711 + (t54 - 0.1e1 * t84) * t683) * t365 + (-0.1e1 * t230 + t736) * t845 + t191 * t683 + (t188 * t374 - t364 * t77 + t568) * t366) * t372 + (t739 * t687 + (t256 * t374 + t286) * t373 + (-0.1e1 * t663 + t40 * t687 + (t186 + t580) * t374 - 0.1e1 * t807) * t366) * t365 - t77 * t688 + ((-0.1e1 * t230 - 0.1e1 * t736) * t364 - 0.66241105529490700000e-2 * t374) * t373 - 0.16444875773692700000e-2 * t700 - 0.1e1 * t182 * t711 + ((-0.1e1 * t765 + 0.2502297872941088000e-2 * t357 + 0.790217436631504e-3 * t714 - 0.48082828567067140000e-2 - 0.1e1 * t670) * t359 + (((-0.1e1 * t600 + (0.4841887557042460e-2 * t363 + 0.55042935974400000000e-3) * t370 + t267) * t371 - 0.5437511053345940e-2) * t365 + (-0.1e1 * t739 + (-0.24444132201840000000e-2 * t366 + 0.12763550042100000000e-2) * t370 + t532) * t371 - 0.1e1 * t229 - 0.1e1 * t364 * t572 + t824) * t372 + (-0.22516878283212450000e-2 - 0.1e1 * t787) * t353 + (-0.1e1 * t254 * t373 - 0.1e1 * t264 - 0.1e1 * t566) * t365 + t526 * t358 + (-0.1e1 * t422 + 0.52863517876992000000e-1) * t371 + (-0.1e1 * t556 * t364 - 0.50330438027992300000e0) * t373 + (0.29682175996164750000e0 + t740) * t366 - 0.1e1 * t755 - 0.65337013765020712700e0) * t367) * t368;
  t2 = ((((t318 + t479 + t817) * t359 + (t364 * t97 - t871 - 0.1e1 * t454) * t372 - 0.1e1 * t121 + (t183 * t364 + 0.52863517876992000000e-1) * t371 - 0.1e1 * t754 + t328 + t531 + t783) * t700 - 0.1e1 * t575 * t711 + (t753 - t770 - 0.1e1 * t186) * t698) * t373 + (t286 * t372 + t340 * t371) * t366 + t807 * t372 - 0.1e1 * t698 * t861 + t365 * t568 + ((((-0.1e1 * t813 + t182) * t371 + t408) * t372 - 0.1e1 * t771 - t872 - 0.1e1 * t540) * t360 + (t740 + t758 - 0.1e1 * t823 + t842) * t373 + (t802 * t372 - 0.1e1 * t746 - 0.1e1 * t147 - 0.58416762559717300000e0) * t366 + t870 * t372 + t498 * t371 + (t199 - t76) * t364 + t750 + 0.36044563611157510600e0) * t374 + (((t303 - 0.1e1 * t443 + t786) * t372 + 0.1644487577369270e-2) * t373 + (-t857 + (-0.1e1 * t314 + 0.55993270925625000000e-2) * t372 + (-0.1e1 * t413 - 0.1e1 * t313) * t371 + (-0.1e1 * t202 + t322) * t364 - 0.6624110552949070e-2 + ((-0.1e1 * t658 + t459) * t372 + t150 - 0.12089329343850000000e-2) * t365) * t366 - 0.1e1 * t516 - 0.13297019103287584000e-1) * t367) * t368 + ((t522 + t819) * t366 - 0.1e1 * t756 + t603) * t682 + t90 * t699 + ((t456 + t783) * t360 + (0.16666470322297176900e0 + t464) * t354 + (t494 + 0.17515606502671400000e-3) * t353 + 0.81354094419858e-4 * t357 + t336 + t794) * t375;
  t1 = (((-0.1e1 * t729 + 0.22900e-3) * t372 + (-0.1e1 * t562 - 0.1e1 * t278 - 0.1e1 * t791) * t365 + t779) * t682 - 0.1e1 * t784 * t661 + t36 * t372 * t655 + t156 * t652 - 0.1e1 * t512 * t699 + (-0.12805000000000000000e-1 + t643 * t366) * t375) * t374 + (t36 * t359 + t858 + t388 - 0.1e1 * t656) * t682 * t703 + t367 * (t428 + 0.414600e-2 + t791) * t684 - 0.1e1 * t213 * t686 * t698 - 0.70400000000000000000e-3 * t375 - 0.3228604e1 * (-0.1e1 * (t172 * t369 + t376 * t467) * t376 - 0.1e1 * t369 * ((-0.1e1 * t843 + t631) * t376 + t467 * t369)) * t171 + (t26 * t360 - 0.19192000000000000000e-1 + (-0.1e1 * t156 * t364 + 0.22900e-3) * t365) * t367 * t375 + ((0.95220000000000000000e-2 + ((-0.1e1 * t764 - 0.84680e-2 + (-0.1e1 * t555 - 0.1e1 * t276) * t364) * t359 + (t126 - 0.1e1 * t122 + t396) * t705 - 0.1e1 * t762 + t287 - 0.1e1 * t782) * t373 + ((-0.1e1 * t730 + 0.45800e-3) * t372 - 0.172820e-1 - 0.1e1 * t394 * t709 + t801 * t365) * t366) * t361 + ((-0.1e1 * t841 + (-0.1e1 * t762 + t536 + t723) * t705 - 0.1e1 * t393 + t679) * t360 + t26 * t701 + (-0.1e1 * t595 + t657 + 0.27049999999999999999e-2 + (t598 + 0.85599999999999999997e-3 * t714) * (-0.1e1 * t358 - 0.1e1)) * t359 + ((-0.49779999999999999999e-2 * t714 + t451) * t371 + (t587 + 0.68199999999999999999e-3) * t364 + t536) * t705 + t830) * t694 - 0.15015000000000000000e-1 + (t156 * t371 - 0.1e1 * t784 * t359 + t36 * t705 - 0.1e1 * t512 + t643) * t373 + ((-0.22900e-3 + t729) * t372 + (-0.1e1 * t731 - 0.1e1 * t660 + t562 + t278) * t365 - 0.1e1 * t779) * t366) * t368 + 0.1666555e1 * (((t818 * t375 + (0.1e1 * t847 - 0.1e1 * t728) * t368) * t369 + (-0.1e1 * t173 * t374 + t367 * t803) * t376) * t376 + ((((-0.1e1 * t846 - 0.1e1 * t215 + 0.825e-1) * t374 - 0.1e1 * t406) * t375 + t609 * t368) * t376 - 0.1e1 * t173 * t689 + 0.1e1 * t826 * t369 * t695 + t207 * t697) * t369) * ((t609 + 0.316e0) * t375 + t818 * t368) + 0.2261006370e-2 * (t868 + 0.1e1 * t869) * t274 + 0.3587895e1 * (-0.1e1 * t868 - 0.1e1 * t869) * (t236 * t367 + 0.27454e-1 * t374) * (-0.1e1 * t368 * t520 + t436) + 0.73552200000000000000e0 * (t376 * ((-t853 + (t373 * t49 + t767) * t374) * t369 * t375 + (-0.1e1 * t125 * t691 + t49 * t692) * t373 + (t49 * t366 - 0.316e0) * t691 + t692 * t767 + ((-0.1e1 * t812 + t844) * t374 - 0.1e1 * t648) * t376) + t369 * ((t51 * t367 + (-0.1e1 * t848 + t865) * t374) * t376 * t375 + (t125 * t690 - 0.1e1 * t65 * t697) * t373 + (t366 * t65 + 0.316e0) * t690 + t51 * t689 + t697 * t848 - 0.1e1 * t369 * t648)) * ((-0.1e1 * t835 * t366 + t89 * t373 + 0.31600000000000000000e0) * t375 + ((-0.1e1 * t216 * t372 + (t579 + t742) * t365) * t367 + (t89 * t366 + t835 * t373 - 0.82500000000000000000e-1) * t374) * t368) + 0.1225946e1 * ((t368 * t502 + t375 * t68 - 0.1e1 * t350) * t369 + t478 * t376) * t376 * (t68 * t368 - 0.1e1 * t806) - 0.1225946e1 * (((t217 * t367 - 0.1e1 * t105) * t375 + t350 + (t628 - 0.1e1 * t727) * t368) * t376 + t478 * t369) * ((-0.1e1 * t105 + t805) * t368 + t806) * t369;
  M(6,6) = t342 + t481;
  M(1,7) = t9;
  M(1,1) = 0.12995663955041442320e1 + (-0.75032996182843272500e0 + ((t670 + t765 + t796) * t359 + (-t371 * t488 + t538) * t705 + t822) * t361 + ((t53 + t790) * t359 + ((-t859 - 0.1e1 * t504) * t371 - t862 - 0.1e1 * t446) * t372 + (-0.2489553776598929990e-3 + t493) * t358 + t775) * t360 + (-0.67903019910400000000e0 + ((t421 + t785) * t372 + ((t718 - 0.1e1 * t308 - 0.1e1 * t334 + 0.5826996021941340000e-3) * t365 + t504) * t364 + t854) * t366) * t373 + ((t329 - 0.1e1 * t484) * t358 - 0.1e1 * t664 + t596 + t419) * t359 + (t499 + t72) * t705 + t53 + t662 + 0.18916511922000000000e0 * t366 - 0.1e1 * t460) * t850 + 0.7678648964878236e-2 * t361 + 0.62964373601650000000e0 * t373 + 0.175156065026714e-3 * t359 + (t163 * t353 - 0.1e1 * t526) * t358 - 0.1e1 * t184 * t715 * t371 + t755 - 0.36644357310000000000e0 * t366 + t320 + ((-0.79667177678710400000e-2 + (0.72089127222315021200e0 + (((-0.13379861294270224000e-1 * t370 + 0.43868728512658559996e-2 * t363 - 0.44088275061402520000e-1) * t358 + ((-0.96305836223205680040e-2 * t357 + (-0.1e1 * t586 + 0.54457813512960000000e-2) * t370 + 0.53191491764352000000e-4 * t351 + 0.22017174389760000000e-2 * t363 + 0.23121910499710648004e-1) * t364 + t397) * t371 + 0.10572703575398400000e0 * t364 + t552 - 0.1e1 * t306 + 0.17936986422585684000e-1) * t372 + (-0.1e1 * t201 * t365 + 0.22714792837770000000e-1) * t371 + (-0.1e1 * t461 * t365 + t398) * t364 + (-0.48037471395840000000e-2 * t370 + 0.11881704766464000000e-1 * t363 - 0.95593081660407480000e-1) * t365 - 0.55505629074184340000e0) * t360 + ((t196 * t371 + 0.43502269919608000000e-1 * t364 - 0.92611589640160000000e-2) * t372 - 0.1e1 * t550 + t804 + t129 - 0.25817947234305000000e-1) * t373 + (t259 * t364 + t421 + t860) * t372 + (t144 + t530) * t371 + t487 * t364 + t752 + ((((-0.1e1 * t341 + t484) * t358 + 0.96165657134134280000e-2 + t390) * t359 + ((((-0.9683775114084920003e-2 * t363 - 0.11008587194880000000e-2) * t370 - 0.11653992043882679999e-2 + t672) * t365 + t398) * t371 + ((0.21934364256329279999e-2 * t370 + t584 + 0.3742763892584200000e-3) * t365 - 0.22714792837770000000e-1) * t364 + 0.10875022106691880e-1 * t365 + 0.48357317375400000000e-2) * t372 + (-0.4841887557042460002e-2 * t357 - 0.1e1 * t283 - 0.4979107553197859980e-3) * t358 + (t180 * t364 + 0.10572703575398400000e0) * t371 + (-0.27228906756480000000e-2 * t370 - 0.1e1 * t310 - 0.12085461751057286000e-1) * t352 - 0.1e1 * t397 * t364 + 0.45033756566424900000e-2 * t353 + (-0.25527100084200000000e-2 * t363 + 0.10320550495200000000e-2 * t370 + 0.22397308370250000000e-1) * t365 + 0.96837751140849200040e-2 * t357 + t370 * t586 - 0.10871993142954728220e1) * t373 + t825 * t372 - 0.1e1 * t743 - 0.1e1 * t756 - 0.11683352511943460000e1) * t366) * t374 + (((-0.1e1 * t718 - 0.1e1 * t521) * t364 + t828) * t372 + (t134 + t785) * t365 + t604) * t695 + ((-0.1e1 * t309 + ((-0.1e1 * t299 - 0.13950377157815110002e-1 - 0.1e1 * t310 + t678) * t358 - 0.1e1 * t665 + 0.5004595745882176002e-2 * t357 + t419) * t365 + t444) * t366 + t433) * t696 + (t101 * t366 - 0.43502269919608000000e-1 * t365) * t711 + 0.92611589640160000000e-2 * t698 + ((-0.1e1 * t72 - 0.1e1 * t499) * t359 - 0.13248221105898140000e-1 - 0.1e1 * t577) * t703 + (((t365 * t504 + t488) * t366 - 0.1e1 * t196 * t365) * t371 - 0.26594038206575168000e-1) * t367) * t375 + ((-0.46255063132042766200e0 + ((-0.1e1 * t53 - 0.1e1 * t790) * t359 + (t371 * t487 + t446 + t862) * t372 + (0.24895537765989299900e-3 - 0.1e1 * t493) * t358 - 0.1e1 * t775) * t360 + (0.49386463087500000000e-1 + ((-0.1e1 * t134 - t860 - 0.1e1 * t312 + t437) * t372 + (t86 * t365 - 0.1e1 * t317 - 0.1e1 * t337 - 0.27219646194675000000e-1) * t364 - t854) * t366) * t373 + (t163 * t358 - 0.1e1 * t662 + 0.22516878283212450000e-2) * t359 - t788 * t358 + t664 + 0.17727845388000000000e0 * t366 + t321 - t838) * t361 + (((t72 + (-0.37427638925842000000e-3 + t425) * t364 - 0.10875022106691880000e-1) * t359 - 0.1e1 * t175 * t372 + t772 - 0.1e1 * t101 * t364 + 0.13248221105898140000e-1 + (((-0.1e1 * t329 + t484) * t358 + 0.51131900567709380000e-2 + t390) * t372 - t825) * t365) * t373 + ((t364 * t86 + t828) * t366 + t175) * t372 + t707 * t134 + (t366 * t645 + t504) * t706 + (-0.52863517876992000000e-1 * t366 + 0.11357396418885000000e-1) * t713 + t604 * t366 - 0.1e1 * t577 + 0.2438248419014880000e-3) * t694 + (-0.43502269919608000000e-1 * t371 + t743 + 0.40844180677309600000e0) * t373 + ((t196 * t366 - 0.1e1 * t504) * t371 + t530 * t364 - 0.92611589640160000000e-2 * t366 + 0.24178658687700000000e-2) * t372 + (t129 - 0.12056561435880000000e0) * t366 + t756 + 0.21165494803694631600e0) * t368) * t368 + (0.76786489648782360000e-2 * t850 + ((0.60294330025875550000e-2 + t300 + t671) * t358 + t318 - 0.1e1 * t298 + t796) * t359 + (t538 + t772) * t705 + t822) * t355;
  M(7,2) = t12;
  M(1,4) = t3;
  M(3,5) = t13;
  M(5,6) = t42;
  M(6,4) = t24;
  M(1,3) = t2;
  M(2,3) = t4;
  M(7,6) = -t430;
  M(5,2) = t8;
  M(1,5) = t5;
  M(6,5) = t42;
  M(7,7) = 0.49096519673609460000e-2;
  M(2,7) = t12;
  M(1,2) = t1;
  M(3,4) = t11;
  M(6,1) = t7;
  M(1,6) = t7;
  M(2,5) = t8;
  M(4,5) = t20;
  M(4,7) = t25;
  M(5,4) = t20;
  M(2,2) = 0.646926e0 * (0.2872e-1 * t368 - 0.3141e-2 * t375) ^ 2 + 0.3587895e1 * (t368 * t469 + t375 * t520 - t350) ^ 2 + (-0.95220e-2 + ((t764 + 0.84680e-2 + (t276 + t555) * t364) * t359 + (-0.1e1 * t396 + t680) * t705 + t669 + t782) * t373 + (0.172820e-1 + (-0.1e1 * t732 - 0.1e1 * t659 + t558 - 0.1e1 * t277) * t365 + t799 * t372) * t366) * t694 + 0.1225946e1 * (t409 * t368 + (-t805 + (t373 * t472 + t290) * t374) * t375 + t651) ^ 2 - 0.1e1 * t595 + t656 + 0.735522e0 * (t384 * t368 + (-t853 + (t366 * t836 + t385 * t373 - 0.825e-1) * t374) * t375 + t623) ^ 2 + (-0.1e1 * t858 + (0.27050000000000000000e-2 + t679 - 0.1e1 * t416) * t359 + t830) * t361 + 0.1666555e1 * (t832 * t368 + (t406 + (t366 * t473 + t373 * t411 - 0.825e-1) * t374) * t375 + t623) ^ 2 + ((t841 + t388 - 0.1e1 * t657 + (-0.1e1 * t723 - 0.42340000000000000000e-2 + t669) * t705) * t360 + (-0.15592000000000000000e-1 + ((-0.43600000000000000000e-3 + t492) * t358 + (-0.56440000000000000000e-2 - 0.1e1 * t415) * t710 + t558 + 0.82920000000000000000e-2 - 0.1e1 * t307) * t372 + ((t426 - 0.68200000000000000000e-3) * t371 + 0.45800000000000000000e-3 + (-0.1e1 * t517 + t451) * t364) * t365) * t701) * t355 + 0.10340700000000000000e0 + 0.3228604e1 * t172 ^ 2 + t416 * t352 + (t868 + t869) * (0.735522e0 * ((-0.316e0 + t384) * t375 + (t853 + (-t848 + t865) * t374) * t368 - t675) ^ 2 + 0.3228604e1 * t171 ^ 2 + 0.1666555e1 * ((0.316e0 - t832) * t375 + (t406 + (t215 + t846) * t374) * t368 + t675) ^ 2 + 0.1225946e1 * (-(-0.316e0 + t409) * t375 - (t805 + (-t345 - t726) * t374) * t368 + t675) ^ 2 + 0.3587895e1 * (t295 + t436 + (t374 * t470 + t637) * t368) ^ 2 + 0.646926e0 * t274 ^ 2);
  M(3,2) = t4;
  M(3,3) = (-t734 + (0.51602752476000000000e-3 * t365 + t589) * t370 + t719 + t456) * t360 + ((0.27752814537092170000e0 + t804 + t819) * t366 - 0.1e1 * t719 + t603 + ((t364 * t93 + t185) * t366 - 0.1e1 * t566) * t365) * t373 + (0.166664703222971769e0 + t464) * t354 + t90 * t366 + (-0.24890000000000000000e-2 * t353 + 0.81354094419858e-4) * t357 + (-t353 * t592 + 0.13614453378240000000e-2) * t370 + t321 + t794;
  M(2,6) = t10;
  M(7,4) = t25;
  M(7,5) = t71;
  M(4,1) = t3;
  M(7,3) = t19;
  M(4,4) = ((t342 + t523) * t358 + t318 - 0.81354094419858e-4 * t351 + t503) * t359 + (-t365 * t38 - t797) * t372 + (0.2251687828321245e-2 + t787) * t353 + t756 + (t343 + 0.1194710953979893e-2) * t358 + t501 + t777;
  M(5,3) = t13;
  M(4,3) = t11;
  M(7,1) = t9;
  M(2,1) = t1;
  M(6,2) = t10;
  M(3,1) = t2;
  M(5,5) = t187 * t358 + t658 + t852;
  M(3,6) = t18;
  M(6,3) = t18;
  M(2,4) = t6;
  M(3,7) = t19;
  M(6,7) = -t430;
  M(4,6) = t24;
  M(5,7) = t71;
  M(4,2) = t6;
  M(5,1) = t5;
end

== matlab function Controller_damping_cbf/Visualisation/MATLAB Function1 ==
  data: H input; d output
function d = fcn(H)

d = H(1:3,4);

end

== matlab function Controller_damping_cbf/Visualisation/MATLAB Function3 ==
  data: wrench input; F_ext output
function F_ext = fcn(wrench)

F_ext = wrench(1:3);


end

== matlab function Controller_damping_cbf/Visualisation/MATLAB Function5 ==
  data: x_ref_dot input; p_ref_dot output
function p_ref_dot = fcn(x_ref_dot)

p_ref_dot = x_ref_dot(1:3);

end

== matlab function Controller_damping_cbf/task space controller/Subsystem4/MATLAB Function ==
  data: q_dot input; V_tilde output; Jg input; V_body_ref input; H_I_t input; H_I_D input
function V_tilde = computePositionError(q_dot, Jg, V_body_ref, H_I_t, H_I_D)

p = Jg*q_dot;

R_I_t = H_I_t(1:3,1:3);
R_I_D = H_I_D(1:3,1:3);

% V_tilde = blkdiag(R_I_t',R_I_t')*( p - blkdiag(R_I_D,R_I_D)*V_body_ref) ;

V_tilde = zeros(6,1);
% V_tilde(1:3) = R_I_t'*p(1:3) - R_I_t'*R_I_D*V_body_ref(1:3);
% V_tilde(4:6) = R_I_t'*p(4:6) - R_I_t'*R_I_D*V_body_ref(4:6);

V_tilde(1:3) = p(1:3) - R_I_D*V_body_ref(1:3);
V_tilde(4:6) = p(4:6) - R_I_D*V_body_ref(4:6);


end

== matlab function Controller_damping_cbf/Visualisation/MATLAB Function6 ==
  data: x_ref_dotdot input; p_ref_dotdot output
function p_ref_dotdot = fcn(x_ref_dotdot)

p_ref_dotdot = x_ref_dotdot(1:3);

end

== matlab function Controller_damping_cbf/Visualisation/MATLAB Function2 ==
  data: H input; angle output; tol input
function angle = Rot2zyxAngles(H, tol)

R = H(1:3,1:3);
angle = zeros(3,1);

if( abs(R(3,1))<= 1-tol )
    angle(1) = atan2(R(2,1),R(1,1));
    angle(2) = atan2(-R(3,1),sqrt( (R(1,1))^2 + (R(2,1))^2 ));
    angle(3) = atan2(R(3,2),R(3,3));
elseif( R(3,1)<= -1+tol )
    angle(1) = 0;
    angle(2) = pi/2;
    angle(3) = atan2(R(1,2),R(2,2));
elseif( 1-tol <= R(3,1))
    angle(1) = 0;
    angle(2) = -pi/2;
    angle(3) = -atan2(R(1,2),R(2,2));
end

end

== matlab function Controller_damping_cbf/task space controller/impedance controller1 ==
  data: F_control output; q_dot input; V_tilde input; V_ref_dot input; massM input; lambdaM input; C input; Jg input; Jg_dot input; JgRightPseu input; Fk input; Dd input; H_I_D input; n_hp input; d_add input
function F_control  = Cartesian_impedance_control(q_dot, V_tilde, V_ref_dot, massM, lambdaM, C, Jg,...
    Jg_dot, JgRightPseu, Fk, Dd, H_I_D, n_hp, d_add)

% Dd = diag(Dd);
R_I_D = H_I_D(1:3,1:3);
V_ref_dot = blkdiag(R_I_D,R_I_D)*V_ref_dot;
v_c = dot(n_hp, V_tilde);



massMInv = massM\eye(7);
massMInv = (massMInv + transpose(massMInv))./2;
mu = lambdaM*(Jg*massMInv*C - Jg_dot);

% Variante 1
F_c = mu*q_dot + lambdaM*V_ref_dot - mu*JgRightPseu*V_tilde - Dd*V_tilde - Fk;
% F = lambdaM*(Jg*massMInv*C - Jg_dot) * (q_dot-JgRightPseu*V_tilde) -Dd*V_tilde - Fk;
% F =  -Dd*V_tilde - Fk;


% Lambda_inv = lambdaM\eye(6);
Lambda_inv = Jg*massMInv*transpose(Jg);
Lambda_inv = (Lambda_inv + transpose(Lambda_inv))./2;

m_c = (transpose(n_hp)*Lambda_inv*n_hp)\eye(1);
C_c = (m_c^2) .*(transpose(n_hp) *Lambda_inv * mu*JgRightPseu * Lambda_inv * n_hp);

% Variante 2
% F_c  =  mu*q_dot + lambdaM*V_ref_dot + (m_c.*(n_hp*transpose(n_hp))*Lambda_inv - eye(6))*(mu*JgRightPseu*V_tilde + Dd*V_tilde + Fk) - (C_c+d_add).*(n_hp*transpose(n_hp)*V_tilde);
F_c2  =  n_hp*( m_c.*(transpose(n_hp)*Lambda_inv)*(mu*JgRightPseu*V_tilde + Dd*V_tilde + Fk)) + n_hp.*(-C_c*v_c - d_add*v_c);




% F_control = F_c + F_c2;
F_control = F_c ;




end
